simulink library "ConverterLibrary"  (R2026a)
settings: Solver=VariableStepAuto
undefined symbols (not defined in the file or in its folder): DiscIntNeverNeededParam, dspblkCoreblockFVToolHelper, gcbh, gridInverter
libraries: fl_lib x240, nesl_utility x221, ee_lib x208, slpidlib x28, eeGeneralControl x12, simulink x9, eeTransforms x4, simulink_extras x1, eePowerMeasurement x1
(part 2 of 30)

== system ConverterLibrary/Controller/PWM Generators ==
  CLLC PWM Generator : Subsystem  mask(CLLC Resonant Converter PWM Generator){solverMode=Variable-step (continuous), Ts=1e-8, Fbase=100e3, fpuMin=0.6, fpuMax=1.55, pulseWidth=0.5, Tdead=250e-9, Ith=0.5, fpuSrLower=0.97, fpuSrUpper=1.03, Tsr=100e-9, gateVoltageOn=15, gateVoltageOff=0, srGateVoltageOn=15, srGateVoltageOff=0}
      mask prompts: solverMode "Solver mode"; Ts "Sample time (s)"; Fbase "Base (resonant) frequency (Hz)"; fpuMin "Minimum normalized frequency (pu)"; fpuMax "Maximum normalized frequency (pu)"; pulseWidth "Pulse width (fraction of switching period)"; Tdead "Dead time (s)"; Ith "Rectifier current threshold (A)"; fpuSrLower "Resonance band lower edge (pu)"; fpuSrUpper "Resonance band upper edge (pu)"; Tsr "Rectifier turn-on delay (s)"; gateVoltageOn "Gate ON voltage (V)"; gateVoltageOff "Gate OFF voltage (V)"; srGateVoltageOn "Rectifier gate ON voltage (V)"; srGateVoltageOff "Rectifier gate OFF voltage (V)"
      mask help:
      | This block generates full-bridge PWM gate signals with a dead time from a commanded switching frequency, and synchronous rectifier gate signals from the rectifier current.
      |
      | Set the rectifier band lower edge below its upper edge. For a variable-step solver, set Solver mode to Variable-step (continuous). For a fixed-step solver, set Solver mode to Fixed-step (discrete) and set Sample time to a positive value.
      mask init:
      | % Solver mode. Switch every sawtooth ramp in this block between its continuous
      | % and its discrete implementation, and show the sample time only when it is used.
      | pwmGeneratorBlock = gcb;
      | if strcmp(get_param(pwmGeneratorBlock, 'solverMode'), 'Fixed-step (discrete)')
      |     pwmGeneratorRampChoice = 'FixedStep';
      |     pwmGeneratorSampleTimeVisibility = 'on';
      | else
      |     pwmGeneratorRampChoice = 'VariableStep';
      |     pwmGeneratorSampleTimeVisibility = 'off';
      | end
      | 
      | % A block may hold more than one ramp, at any depth, so the ramps are found by the
      | % "Ramp Mode" suffix on their names rather than by one fixed path. The match filter
      | % keeps every variant choice in the search, which is also what silences the
      | % find_system default-variants warning.
      | pwmGeneratorRamps = find_system(pwmGeneratorBlock, ...
      |     'MatchFilter', @Simulink.match.allVariants, 'LookUnderMasks', 'all', ...
      |     'FollowLinks', 'on', 'Regexp', 'on', 'BlockType', 'SubSystem', ...
      |     'Name', 'Ramp Mode$');
      | for pwmGeneratorRampIndex = 1:numel(pwmGeneratorRamps)
      |     set_param(pwmGeneratorRamps{pwmGeneratorRampIndex}, ...
      |         'LabelModeActiveChoice', pwmGeneratorRampChoice);
      | end
      | 
      | % Only the discrete ramp declares a rate, so the sample time is hidden in the
      | % continuous mode. The guard keeps the code silent on a mask still being built.
      | pwmGeneratorMask = Simulink.Mask.get(pwmGeneratorBlock);
      | pwmGeneratorSampleTime = pwmGeneratorMask.getParameter('Ts');
      | if ~isempty(pwmGeneratorSampleTime)
      |     pwmGeneratorSampleTime.Visible = pwmGeneratorSampleTimeVisibility;
      | end
      mask Help: web('CLLCPWMGenerator.html')
      mask TypeOptions solverMode: Variable-step (continuous) | Fixed-step (discrete)
      mask Callback solverMode:
      | % Solver mode. Switch every sawtooth ramp in this block between its continuous
      | % and its discrete implementation, and show the sample time only when it is used.
      | pwmGeneratorBlock = gcb;
      | if strcmp(get_param(pwmGeneratorBlock, 'solverMode'), 'Fixed-step (discrete)')
      |     pwmGeneratorRampChoice = 'FixedStep';
      |     pwmGeneratorSampleTimeVisibility = 'on';
      | else
      |     pwmGeneratorRampChoice = 'VariableStep';
      |     pwmGeneratorSampleTimeVisibility = 'off';
      | end
      | 
      | % A block may hold more than one ramp, at any depth, so the ramps are found by the
      | % "Ramp Mode" suffix on their names rather than by one fixed path. The match filter
      | % keeps every variant choice in the search, which is also what silences the
      | % find_system default-variants warning.
      | pwmGeneratorRamps = find_system(pwmGeneratorBlock, ...
      |     'MatchFilter', @Simulink.match.allVariants, 'LookUnderMasks', 'all', ...
      |     'FollowLinks', 'on', 'Regexp', 'on', 'BlockType', 'SubSystem', ...
      |     'Name', 'Ramp Mode$');
      | for pwmGeneratorRampIndex = 1:numel(pwmGeneratorRamps)
      |     set_param(pwmGeneratorRamps{pwmGeneratorRampIndex}, ...
      |         'LabelModeActiveChoice', pwmGeneratorRampChoice);
      | end
      | 
      | % Only the discrete ramp declares a rate, so the sample time is hidden in the
      | % continuous mode. The guard keeps the code silent on a mask still being built.
      | pwmGeneratorMask = Simulink.Mask.get(pwmGeneratorBlock);
      | pwmGeneratorSampleTime = pwmGeneratorMask.getParameter('Ts');
      | if ~isempty(pwmGeneratorSampleTime)
      |     pwmGeneratorSampleTime.Visible = pwmGeneratorSampleTimeVisibility;
      | end
      mask DialogControl DescTextVar Prompt:
      | This block generates full-bridge PWM gate signals with a dead time from a commanded switching frequency, and synchronous rectifier gate signals from the rectifier current.
      | 
      | Set the rectifier band lower edge below its upper edge. For a variable-step solver, set Solver mode to Variable-step (continuous). For a fixed-step solver, set Solver mode to Fixed-step (discrete) and set Sample time to a positive value.
      mask DialogControl SolverPanel Prompt: Solver Settings
      mask DialogControl SwitchingPanel Prompt: Switching Parameters
      mask DialogControl SyncRectifierPanel Prompt: Synchronous Rectifier
      mask DialogControl GateDrivePanel Prompt: Gate Drive
  Complementary PWM Generator : Subsystem  mask(Complementary PWM Generator){solverMode=Variable-step (continuous), Ts=1e-8, Tdead=100e-9, inputLogicThreshold=0.5, gateVoltageOn=15, gateVoltageOff=0}
      mask prompts: solverMode "Solver mode"; Ts "Sample time (s)"; Tdead "Dead time (s)"; inputLogicThreshold "Input logic threshold (V)"; gateVoltageOn "Gate ON voltage (V)"; gateVoltageOff "Gate OFF voltage (V)"
      mask help:
      | This block splits one PWM signal into a complementary gate pair with a dead time.
      |
      | For a variable-step solver, set Solver mode to Variable-step (continuous). For a fixed-step solver, set Solver mode to Fixed-step (discrete) and set Sample time to a positive value.
      mask init: same as ConverterLibrary/Controller/PWM Generators/CLLC PWM Generator
      mask Help: web('ComplementaryPWMGenerator.html')
      mask TypeOptions solverMode: Variable-step (continuous) | Fixed-step (discrete)
      mask Callback solverMode:
      | % Solver mode. Switch every sawtooth ramp in this block between its continuous
      | % and its discrete implementation, and show the sample time only when it is used.
      | pwmGeneratorBlock = gcb;
      | if strcmp(get_param(pwmGeneratorBlock, 'solverMode'), 'Fixed-step (discrete)')
      |     pwmGeneratorRampChoice = 'FixedStep';
      |     pwmGeneratorSampleTimeVisibility = 'on';
      | else
      |     pwmGeneratorRampChoice = 'VariableStep';
      |     pwmGeneratorSampleTimeVisibility = 'off';
      | end
      | 
      | % A block may hold more than one ramp, at any depth, so the ramps are found by the
      | % "Ramp Mode" suffix on their names rather than by one fixed path. The match filter
      | % keeps every variant choice in the search, which is also what silences the
      | % find_system default-variants warning.
      | pwmGeneratorRamps = find_system(pwmGeneratorBlock, ...
      |     'MatchFilter', @Simulink.match.allVariants, 'LookUnderMasks', 'all', ...
      |     'FollowLinks', 'on', 'Regexp', 'on', 'BlockType', 'SubSystem', ...
      |     'Name', 'Ramp Mode$');
      | for pwmGeneratorRampIndex = 1:numel(pwmGeneratorRamps)
      |     set_param(pwmGeneratorRamps{pwmGeneratorRampIndex}, ...
      |         'LabelModeActiveChoice', pwmGeneratorRampChoice);
      | end
      | 
      | % Only the discrete ramp declares a rate, so the sample time is hidden in the
      | % continuous mode. The guard keeps the code silent on a mask still being built.
      | pwmGeneratorMask = Simulink.Mask.get(pwmGeneratorBlock);
      | pwmGeneratorSampleTime = pwmGeneratorMask.getParameter('Ts');
      | if ~isempty(pwmGeneratorSampleTime)
      |     pwmGeneratorSampleTime.Visible = pwmGeneratorSampleTimeVisibility;
      | end
      mask DialogControl DescTextVar Prompt:
      | This block splits one PWM signal into a complementary gate pair with a dead time.
      | 
      | For a variable-step solver, set Solver mode to Variable-step (continuous). For a fixed-step solver, set Solver mode to Fixed-step (discrete) and set Sample time to a positive value.
      mask DialogControl SolverPanel Prompt: Solver Settings
      mask DialogControl SwitchingPanel Prompt: Switching Parameters
      mask DialogControl GateDrivePanel Prompt: Gate Drive
  DAB PWM Generator : Subsystem  mask(Dual Active Bridge PWM Generator){solverMode=Variable-step (continuous), Ts=1e-8, Fsw=100e3, Tdead=100e-9, primaryGateVoltageOn=15, primaryGateVoltageOff=0, secondaryGateVoltageOn=15, secondaryGateVoltageOff=0}
      mask prompts: solverMode "Solver mode"; Ts "Sample time (s)"; Fsw "Switching frequency (Hz)"; Tdead "Dead time (s)"; primaryGateVoltageOn "Primary bridge gate ON voltage (V)"; primaryGateVoltageOff "Primary bridge gate OFF voltage (V)"; secondaryGateVoltageOn "Secondary bridge gate ON voltage (V)"; secondaryGateVoltageOff "Secondary bridge gate OFF voltage (V)"
      mask help:
      | This block generates dual-active-bridge PWM gate signals with a dead time from a commanded phase shift.
      |
      | For a variable-step solver, set Solver mode to Variable-step (continuous). For a fixed-step solver, set Solver mode to Fixed-step (discrete) and set Sample time to a positive value.
      mask init: same as ConverterLibrary/Controller/PWM Generators/CLLC PWM Generator
      mask Help: web('DABPWMGenerator.html')
      mask TypeOptions solverMode: Variable-step (continuous) | Fixed-step (discrete)
      mask Callback solverMode:
      | % Solver mode. Switch every sawtooth ramp in this block between its continuous
      | % and its discrete implementation, and show the sample time only when it is used.
      | pwmGeneratorBlock = gcb;
      | if strcmp(get_param(pwmGeneratorBlock, 'solverMode'), 'Fixed-step (discrete)')
      |     pwmGeneratorRampChoice = 'FixedStep';
      |     pwmGeneratorSampleTimeVisibility = 'on';
      | else
      |     pwmGeneratorRampChoice = 'VariableStep';
      |     pwmGeneratorSampleTimeVisibility = 'off';
      | end
      | 
      | % A block may hold more than one ramp, at any depth, so the ramps are found by the
      | % "Ramp Mode" suffix on their names rather than by one fixed path. The match filter
      | % keeps every variant choice in the search, which is also what silences the
      | % find_system default-variants warning.
      | pwmGeneratorRamps = find_system(pwmGeneratorBlock, ...
      |     'MatchFilter', @Simulink.match.allVariants, 'LookUnderMasks', 'all', ...
      |     'FollowLinks', 'on', 'Regexp', 'on', 'BlockType', 'SubSystem', ...
      |     'Name', 'Ramp Mode$');
      | for pwmGeneratorRampIndex = 1:numel(pwmGeneratorRamps)
      |     set_param(pwmGeneratorRamps{pwmGeneratorRampIndex}, ...
      |         'LabelModeActiveChoice', pwmGeneratorRampChoice);
      | end
      | 
      | % Only the discrete ramp declares a rate, so the sample time is hidden in the
      | % continuous mode. The guard keeps the code silent on a mask still being built.
      | pwmGeneratorMask = Simulink.Mask.get(pwmGeneratorBlock);
      | pwmGeneratorSampleTime = pwmGeneratorMask.getParameter('Ts');
      | if ~isempty(pwmGeneratorSampleTime)
      |     pwmGeneratorSampleTime.Visible = pwmGeneratorSampleTimeVisibility;
      | end
      mask DialogControl DescTextVar Prompt:
      | This block generates dual-active-bridge PWM gate signals with a dead time from a commanded phase shift.
      | 
      | For a variable-step solver, set Solver mode to Variable-step (continuous). For a fixed-step solver, set Solver mode to Fixed-step (discrete) and set Sample time to a positive value.
      mask DialogControl SolverPanel Prompt: Solver Settings
      mask DialogControl SwitchingPanel Prompt: Switching Parameters
      mask DialogControl GateDrivePanel Prompt: Gate Drive
  Full Bridge PWM Generator : Subsystem  mask(Full Bridge PWM Generator){solverMode=Variable-step (continuous), Ts=1e-8, Fsw=100e3, Tdead=100e-9, gateVoltageOn=15, gateVoltageOff=0}
      mask prompts: solverMode "Solver mode"; Ts "Sample time (s)"; Fsw "Switching frequency (Hz)"; Tdead "Dead time (s)"; gateVoltageOn "Gate ON voltage (V)"; gateVoltageOff "Gate OFF voltage (V)"
      mask help:
      | This block generates full-bridge PWM gate signals with a dead time from a commanded duty cycle.
      |
      | For a variable-step solver, set Solver mode to Variable-step (continuous). For a fixed-step solver, set Solver mode to Fixed-step (discrete) and set Sample time to a positive value.
      mask init: same as ConverterLibrary/Controller/PWM Generators/CLLC PWM Generator
      mask Help: web('FullBridgePWMGenerator.html')
      mask TypeOptions solverMode: Variable-step (continuous) | Fixed-step (discrete)
      mask Callback solverMode:
      | % Solver mode. Switch every sawtooth ramp in this block between its continuous
      | % and its discrete implementation, and show the sample time only when it is used.
      | pwmGeneratorBlock = gcb;
      | if strcmp(get_param(pwmGeneratorBlock, 'solverMode'), 'Fixed-step (discrete)')
      |     pwmGeneratorRampChoice = 'FixedStep';
      |     pwmGeneratorSampleTimeVisibility = 'on';
      | else
      |     pwmGeneratorRampChoice = 'VariableStep';
      |     pwmGeneratorSampleTimeVisibility = 'off';
      | end
      | 
      | % A block may hold more than one ramp, at any depth, so the ramps are found by the
      | % "Ramp Mode" suffix on their names rather than by one fixed path. The match filter
      | % keeps every variant choice in the search, which is also what silences the
      | % find_system default-variants warning.
      | pwmGeneratorRamps = find_system(pwmGeneratorBlock, ...
      |     'MatchFilter', @Simulink.match.allVariants, 'LookUnderMasks', 'all', ...
      |     'FollowLinks', 'on', 'Regexp', 'on', 'BlockType', 'SubSystem', ...
      |     'Name', 'Ramp Mode$');
      | for pwmGeneratorRampIndex = 1:numel(pwmGeneratorRamps)
      |     set_param(pwmGeneratorRamps{pwmGeneratorRampIndex}, ...
      |         'LabelModeActiveChoice', pwmGeneratorRampChoice);
      | end
      | 
      | % Only the discrete ramp declares a rate, so the sample time is hidden in the
      | % continuous mode. The guard keeps the code silent on a mask still being built.
      | pwmGeneratorMask = Simulink.Mask.get(pwmGeneratorBlock);
      | pwmGeneratorSampleTime = pwmGeneratorMask.getParameter('Ts');
      | if ~isempty(pwmGeneratorSampleTime)
      |     pwmGeneratorSampleTime.Visible = pwmGeneratorSampleTimeVisibility;
      | end
      mask DialogControl DescTextVar Prompt:
      | This block generates full-bridge PWM gate signals with a dead time from a commanded duty cycle.
      | 
      | For a variable-step solver, set Solver mode to Variable-step (continuous). For a fixed-step solver, set Solver mode to Fixed-step (discrete) and set Sample time to a positive value.
      mask DialogControl SolverPanel Prompt: Solver Settings
      mask DialogControl SwitchingPanel Prompt: Switching Parameters
      mask DialogControl GateDrivePanel Prompt: Gate Drive
  Half Bridge PWM Generator : Subsystem  mask(Half Bridge PWM Generator){solverMode=Variable-step (continuous), Ts=1e-8, Fsw=100e3, Tdead=100e-9, gateVoltageOn=15, gateVoltageOff=0}
      mask prompts: solverMode "Solver mode"; Ts "Sample time (s)"; Fsw "Switching frequency (Hz)"; Tdead "Dead time (s)"; gateVoltageOn "Gate ON voltage (V)"; gateVoltageOff "Gate OFF voltage (V)"
      mask help:
      | This block generates half-bridge PWM gate signals with a dead time from a commanded duty cycle.
      |
      | For a variable-step solver, set Solver mode to Variable-step (continuous). For a fixed-step solver, set Solver mode to Fixed-step (discrete) and set Sample time to a positive value.
      mask init: same as ConverterLibrary/Controller/PWM Generators/CLLC PWM Generator
      mask Help: web('HalfBridgePWMGenerator.html')
      mask TypeOptions solverMode: Variable-step (continuous) | Fixed-step (discrete)
      mask Callback solverMode:
      | % Solver mode. Switch every sawtooth ramp in this block between its continuous
      | % and its discrete implementation, and show the sample time only when it is used.
      | pwmGeneratorBlock = gcb;
      | if strcmp(get_param(pwmGeneratorBlock, 'solverMode'), 'Fixed-step (discrete)')
      |     pwmGeneratorRampChoice = 'FixedStep';
      |     pwmGeneratorSampleTimeVisibility = 'on';
      | else
      |     pwmGeneratorRampChoice = 'VariableStep';
      |     pwmGeneratorSampleTimeVisibility = 'off';
      | end
      | 
      | % A block may hold more than one ramp, at any depth, so the ramps are found by the
      | % "Ramp Mode" suffix on their names rather than by one fixed path. The match filter
      | % keeps every variant choice in the search, which is also what silences the
      | % find_system default-variants warning.
      | pwmGeneratorRamps = find_system(pwmGeneratorBlock, ...
      |     'MatchFilter', @Simulink.match.allVariants, 'LookUnderMasks', 'all', ...
      |     'FollowLinks', 'on', 'Regexp', 'on', 'BlockType', 'SubSystem', ...
      |     'Name', 'Ramp Mode$');
      | for pwmGeneratorRampIndex = 1:numel(pwmGeneratorRamps)
      |     set_param(pwmGeneratorRamps{pwmGeneratorRampIndex}, ...
      |         'LabelModeActiveChoice', pwmGeneratorRampChoice);
      | end
      | 
      | % Only the discrete ramp declares a rate, so the sample time is hidden in the
      | % continuous mode. The guard keeps the code silent on a mask still being built.
      | pwmGeneratorMask = Simulink.Mask.get(pwmGeneratorBlock);
      | pwmGeneratorSampleTime = pwmGeneratorMask.getParameter('Ts');
      | if ~isempty(pwmGeneratorSampleTime)
      |     pwmGeneratorSampleTime.Visible = pwmGeneratorSampleTimeVisibility;
      | end
      mask DialogControl DescTextVar Prompt:
      | This block generates half-bridge PWM gate signals with a dead time from a commanded duty cycle.
      | 
      | For a variable-step solver, set Solver mode to Variable-step (continuous). For a fixed-step solver, set Solver mode to Fixed-step (discrete) and set Sample time to a positive value.
      mask DialogControl SolverPanel Prompt: Solver Settings
      mask DialogControl SwitchingPanel Prompt: Switching Parameters
      mask DialogControl GateDrivePanel Prompt: Gate Drive
  LLC PWM Generator : Subsystem  mask(LLC Resonant Converter PWM Generator){solverMode=Variable-step (continuous), Ts=1e-8, Fbase=100e3, fpuMin=0.5, fpuMax=2, pulseWidth=0.5, Tdead=100e-9, gateVoltageOn=15, gateVoltageOff=0}
      mask prompts: solverMode "Solver mode"; Ts "Sample time (s)"; Fbase "Base (resonant) frequency (Hz)"; fpuMin "Minimum normalized frequency (pu)"; fpuMax "Maximum normalized frequency (pu)"; pulseWidth "Pulse width (fraction of switching period)"; Tdead "Dead time (s)"; gateVoltageOn "Gate ON voltage (V)"; gateVoltageOff "Gate OFF voltage (V)"
      mask help:
      | This block generates full-bridge PWM gate signals with a dead time from a commanded switching frequency.
      |
      | For a variable-step solver, set Solver mode to Variable-step (continuous). For a fixed-step solver, set Solver mode to Fixed-step (discrete) and set Sample time to a positive value.
      mask init: same as ConverterLibrary/Controller/PWM Generators/CLLC PWM Generator
      mask Help: web('LLCPWMGenerator.html')
      mask TypeOptions solverMode: Variable-step (continuous) | Fixed-step (discrete)
      mask Callback solverMode:
      | % Solver mode. Switch every sawtooth ramp in this block between its continuous
      | % and its discrete implementation, and show the sample time only when it is used.
      | pwmGeneratorBlock = gcb;
      | if strcmp(get_param(pwmGeneratorBlock, 'solverMode'), 'Fixed-step (discrete)')
      |     pwmGeneratorRampChoice = 'FixedStep';
      |     pwmGeneratorSampleTimeVisibility = 'on';
      | else
      |     pwmGeneratorRampChoice = 'VariableStep';
      |     pwmGeneratorSampleTimeVisibility = 'off';
      | end
      | 
      | % A block may hold more than one ramp, at any depth, so the ramps are found by the
      | % "Ramp Mode" suffix on their names rather than by one fixed path. The match filter
      | % keeps every variant choice in the search, which is also what silences the
      | % find_system default-variants warning.
      | pwmGeneratorRamps = find_system(pwmGeneratorBlock, ...
      |     'MatchFilter', @Simulink.match.allVariants, 'LookUnderMasks', 'all', ...
      |     'FollowLinks', 'on', 'Regexp', 'on', 'BlockType', 'SubSystem', ...
      |     'Name', 'Ramp Mode$');
      | for pwmGeneratorRampIndex = 1:numel(pwmGeneratorRamps)
      |     set_param(pwmGeneratorRamps{pwmGeneratorRampIndex}, ...
      |         'LabelModeActiveChoice', pwmGeneratorRampChoice);
      | end
      | 
      | % Only the discrete ramp declares a rate, so the sample time is hidden in the
      | % continuous mode. The guard keeps the code silent on a mask still being built.
      | pwmGeneratorMask = Simulink.Mask.get(pwmGeneratorBlock);
      | pwmGeneratorSampleTime = pwmGeneratorMask.getParameter('Ts');
      | if ~isempty(pwmGeneratorSampleTime)
      |     pwmGeneratorSampleTime.Visible = pwmGeneratorSampleTimeVisibility;
      | end
      mask DialogControl DescTextVar Prompt:
      | This block generates full-bridge PWM gate signals with a dead time from a commanded switching frequency.
      | 
      | For a variable-step solver, set Solver mode to Variable-step (continuous). For a fixed-step solver, set Solver mode to Fixed-step (discrete) and set Sample time to a positive value.
      mask DialogControl SolverPanel Prompt: Solver Settings
      mask DialogControl SwitchingPanel Prompt: Switching Parameters
      mask DialogControl GateDrivePanel Prompt: Gate Drive

== system ConverterLibrary/Controller/Power Factor Correction Converters ==
  Boost PFC Controller : Subsystem  mask(Boost PFC Controller){outputSelect=PWM Signal, cntrlSelect=PI controller (Continuous), VacRMS=230, VbaseDC=400, Pbase=1000, PrefPu=1, iRefPeakMaxPu=1.3, Fsw=65000, Ts=7.6923e-8, gateVoltageOn=15, gateVoltageOff=0, KpVoltage=1.0392, KiVoltage=11.3097, TsVoltage=7.6923e-6, KpCurrent=0.2602, KiCurrent=3068.1596, dutyMax=0.9935, dutyMin=0.0065, TsCurrent=1.5385e-6}
      mask prompts: outputSelect "Output"; cntrlSelect "Controller type"; VacRMS "Nominal line voltage, RMS (V)"; VbaseDC "Regulated bus voltage (V)"; Pbase "Rated power (W)"; PrefPu "Power command (pu)"; iRefPeakMaxPu "Peak current limit (pu)"; Fsw "Switching frequency (Hz)"; Ts "Modulator sample time (s)"; gateVoltageOn "Gate voltage, on (V)"; gateVoltageOff "Gate voltage, off (V)"; KpVoltage "Voltage-loop proportional gain (pu)"; KiVoltage "Voltage-loop integral gain (pu/s)"; TsVoltage "Voltage-loop sample time (s)"; KpCurrent "Current-loop proportional gain (pu)"; KiCurrent "Current-loop integral gain (pu/s)"; dutyMax "Maximum duty cycle"; dutyMin "Minimum duty cycle"; TsCurrent "Current-loop sample time (s)"
      mask help: Average-current-mode power factor correction controller for the single-leg boost PFC. Regulates the DC bus voltage while shaping the AC line current sinusoidal and in phase, for near-unity power factor. Offers PI controllers in continuous or discrete form, with selectable duty cycle or PWM gate signal output.
      mask init:
      | VbaseAC = sqrt(2)*VacRMS;
      | IbaseAC = 2*Pbase/VbaseAC;
      | VacPeakPuDC = VbaseAC/VbaseDC;
      | 
      | boostPFCControllerMaskInit(gcb);
      mask Help: web('BoostPFCController.html')
      mask TypeOptions outputSelect: Duty Cycle | PWM Signal
      mask Callback outputSelect: boostPFCControllerMaskInit(gcb);
      mask TypeOptions cntrlSelect: PI controller (Continuous) | PI controller (Discrete)
      mask Callback cntrlSelect: boostPFCControllerMaskInit(gcb);
      mask DialogControl ConverterPanel Prompt: Boost PFC Controller Parameters
      mask DialogControl VoltageLoopPanel Prompt: Voltage Controller
      mask DialogControl CurrentLoopPanel Prompt: Current Controller
  Interleaved Boost PFC Controller : Subsystem  mask(Interleaved Boost PFC Controller){outputSelect=PWM Signal, cntrlSelect=PI controller (Continuous), VacRMS=230, VbaseDC=400, Pbase=2000, numberOfLegs=2, PrefPu=1, iRefPeakMaxPu=1.3, Fsw=65000, Ts=7.6923e-8, gateVoltageOn=15, gateVoltageOff=0, KpVoltage=1.0392, KiVoltage=11.3097, TsVoltage=7.6923e-6, KpCurrent=0.2602, KiCurrent=3068.1596, dutyMax=0.9935, dutyMin=0.0065, TsCurrent=1.5385e-6, KpBalance=0.1041, KiBalance=245.4528, dutyBalanceMax=0.1}
      mask prompts: outputSelect "Output"; cntrlSelect "Controller type"; VacRMS "Nominal line voltage, RMS (V)"; VbaseDC "Regulated bus voltage (V)"; Pbase "Rated power (W)"; numberOfLegs "Number of interleaved legs"; PrefPu "Power command (pu)"; iRefPeakMaxPu "Peak current-reference limit (pu)"; Fsw "Switching frequency (Hz)"; Ts "Modulator sample time (s)"; gateVoltageOn "Gate voltage, on (V)"; gateVoltageOff "Gate voltage, off (V)"; KpVoltage "Voltage-loop proportional gain (pu)"; KiVoltage "Voltage-loop integral gain (pu/s)"; TsVoltage "Voltage-loop sample time (s)"; KpCurrent "Current-loop proportional gain (pu)"; KiCurrent "Current-loop integral gain (pu/s)"; dutyMax "Maximum duty cycle"; dutyMin "Minimum duty cycle"; TsCurrent "Current-loop sample time (s)"; KpBalance "Balance-loop proportional gain (pu)"; KiBalance "Balance-loop integral gain (pu/s)"; dutyBalanceMax "Balance-loop duty trim limit"
      mask help: Average-current-mode power factor correction controller for the interleaved boost PFC. Regulates the DC bus voltage while shaping the AC line current sinusoidal and in phase, for near-unity power factor. One shared control serves all legs, with phase-shifted carriers and a differential loop that balances the leg currents. Offers PI controllers in continuous or discrete form, with selectable duty cycle or PWM gate signal output.
      mask init:
      | VbaseAC = sqrt(2)*VacRMS;
      | IbaseAC = 2*Pbase/VbaseAC;
      | VacPeakPuDC = VbaseAC/VbaseDC;
      | 
      | interleavedPFCControllerMaskInit(gcb);
      mask Help: web('InterleavedBoostPFCController.html')
      mask TypeOptions outputSelect: Duty Cycle | PWM Signal
      mask Callback outputSelect: interleavedPFCControllerMaskInit(gcb);
      mask TypeOptions cntrlSelect: PI controller (Continuous) | PI controller (Discrete)
      mask Callback cntrlSelect: interleavedPFCControllerMaskInit(gcb);
      mask DialogControl ConverterPanel Prompt: Interleaved Boost PFC Controller Parameters
      mask DialogControl VoltageLoopPanel Prompt: Voltage Controller
      mask DialogControl CurrentLoopPanel Prompt: Current Controller
      mask DialogControl CurrentBalancePanel Prompt: Current Balance Controller
  Totem-Pole Boost PFC Controller : Subsystem  mask(Totem-Pole Boost PFC Current-Mode Controller){outputSelect=PWM Signal, cntrlSelect=PI controller (Continuous), VacRMS=230, VbaseDC=400, Pbase=3000, Fsw=100000, Fline=50, fastLegDeadTime=1e-07, slowLegTurnOnDelay=0.0001, PrefPu=0.5, iRefPeakMaxPu=1.2, gateVoltageOn=15, gateVoltageOff=0, KpVoltage=1.0392, KiVoltage=11.3097, TsVoltage=5e-06, KpCurrent=0.2602, KiCurrent=4720.2456, dutyMax=1, dutyMin=0, TsCurrent=1e-06}
      mask prompts: outputSelect "Output mode"; cntrlSelect "Controller type"; VacRMS "Nominal AC voltage (V RMS)"; VbaseDC "Nominal DC voltage (V)"; Pbase "Nominal power (W)"; Fsw "Switching frequency (Hz)"; Fline "Line frequency (Hz)"; fastLegDeadTime "Fast-leg dead time (s)"; slowLegTurnOnDelay "Slow-leg turn-on delay (s)"; PrefPu "Feedforward power (pu)"; iRefPeakMaxPu "Peak current limit (pu)"; gateVoltageOn "Gate ON voltage (V)"; gateVoltageOff "Gate OFF voltage (V)"; KpVoltage "Proportional gain (pu)"; KiVoltage "Integral gain (pu/s)"; TsVoltage "Sample time (s)"; KpCurrent "Proportional gain (pu)"; KiCurrent "Integral gain (pu/s)"; dutyMax "Maximum duty cycle"; dutyMin "Minimum duty cycle"; TsCurrent "Sample time (s)"
      mask help: Average-current-mode power factor correction controller for the totem-pole boost PFC. Regulates the DC bus voltage while shaping the AC line current sinusoidal and in phase, for near-unity power factor. Offers PI controllers in continuous or discrete form, with selectable duty cycle or PWM gate signal output.
      mask init:
      | VbaseAC = sqrt(2)*VacRMS;
      | IbaseAC = 2*Pbase/VbaseAC;
      | VacPeakPuDC = VbaseAC/VbaseDC;
      | 
      | totemPolePFCControllerMaskInit(gcb);
      mask Help: web('TotemPoleBoostPFCController.html')
      mask TypeOptions outputSelect: Duty Cycle | PWM Signal
      mask Callback outputSelect: totemPolePFCControllerMaskInit(gcb);
      mask TypeOptions cntrlSelect: PI controller (Continuous) | PI controller (Discrete)
      mask Callback cntrlSelect: totemPolePFCControllerMaskInit(gcb);
      mask DialogControl ConverterPanel Prompt: Totem-Pole Boost PFC Controller Parameters
      mask DialogControl VoltageLoopPanel Prompt: Voltage Controller
      mask DialogControl CurrentLoopPanel Prompt: Current Controller

== system ConverterLibrary/Controller/Soft-Switching Converters ==
  CLLC Controller : Subsystem  mask(CLLC Resonant Converter Voltage Controller){controllerDomain=Continuous, resFreq=100000, ratedPower=10000, Fmin=0.6, Fmax=2.015, Tdead=2.5e-07, VdcValue=400, Kpv=11, Kiv=5500, Kid=0, IdcMax=2.5, IdcMin=-2.5, cntrlSelect=PI controller, Kc=1, numSdomain=[1 1463 1794700], denSdomain=[1 2748.6 0], numZdomain=[1 -1.9985 0.9985], denZdomain=[1 -1.9973 0.9973], Kp=3.5, Ki=5, Ith=0.5, Ibw=300000, vcoSelect=Constant rate, vcoGain=1, vcoGainVec=[1 1.2], pwmSampleTime=1.25e-07, TsVoltage=1e-06, TsCurrent=1e-06}
      mask prompts: controllerDomain "Controller time domain"; resFreq "Resonant frequency"; ratedPower "Rated power (W)"; Fmin "Minimum operating frequency (pu)"; Fmax "Maximum operating frequency (pu)"; Tdead "dead time (s)"; VdcValue "Nominal DC bus voltage"; Kpv "Proportional gain"; Kiv "Integrator gain"; Kid "Differentiator gain"; IdcMax "Maximum output current (pu)"; IdcMin "Minimum output current (put)"; cntrlSelect "Controller type"; Kc "Compensator gain"; numSdomain "Numerator (S domain)"; denSdomain "Denominator (S domain)"; numZdomain "Numerator (Z domain)"; denZdomain "Denominator (Z domain)"; Kp "Proportional gain"; Ki "Integrator gain (Ki)"; Ith "Current threshold (A)"; Ibw "Measurement bandwidth (Hz)"; vcoSelect "Voltage-controlled oscillator type"; vcoGain "VCO gain rate (V/perunit frequency)"; vcoGainVec "VCO gain [g1 g2]  (V/perunit frequency)"; pwmSampleTime "PWM sample time (s)"; TsVoltage "Sample time (s)"; TsCurrent "Sample time (s)"
      mask help: The CLLC resonant converter controller offers four controller options: you can choose between a two-pole, two-zero (2P2Z) compensator and a PI controller, each available in continuous or discrete form. The controller also provides three options for selecting the voltage-controlled oscillator (VCO) gain.
      mask init:
      | % Rate of the block that gates the voltage loop. A discrete voltage controller cannot
      | % inherit a continuous rate, so that block is given the controller rate.
      | gatingSampleTime = gatingSampleTimeForControllerType(controllerDomain, TsVoltage);
      | 
      | cllcControllerMaskInitialization(gcb);
      mask Help: web('CLLCController.html')
      mask TypeOptions controllerDomain: Continuous | Discrete
      mask Callback controllerDomain: selectCLLCControllerVariants(gcb);
      mask TypeOptions cntrlSelect: 2P2Z compensator | PI controller
      mask Callback cntrlSelect: selectCLLCMaskController(gcb);
      mask TypeOptions vcoSelect: Constant rate | Two rate
      mask Callback vcoSelect: selectCLLCControllerMaskVCO(gcb);
      mask DialogControl ParameterGroupVar Prompt: LLC Controller Parameters
      mask DialogControl Container6 Prompt: Voltage Controller Parameters
      mask DialogControl Container3 Prompt: Current Controller Parameters
      mask DialogControl Container5 Prompt: Synchronous rectitifer
      mask DialogControl Container4 Prompt: Voltage-Controlled Oscillator Parameters
      mask DialogControl Container7 Prompt: PWM Generator
  DAB Controller (SPS) : Subsystem  mask(Dual Active Bridge Phase-Shift Controller){outputSelect=Gate Signals, cntrlSelect=PI controller (Continuous), Vbase=525, Pbase=10000, Fsw=100000, Tdead=4.3943e-7, primaryGateVoltage=15, secondaryGateVoltage=15, Ts=1e-07, phaseShiftMax=pi/2, phaseShiftMin=-pi/2, Kp=0.0008, Ki=600, Kpv=0.0075, Kiv=600}
      mask prompts: outputSelect "Output mode"; cntrlSelect "Controller type"; Vbase "Nominal output voltage (V)"; Pbase "Nominal power (W)"; Fsw "Switching frequency (Hz)"; Tdead "Dead time (s)"; primaryGateVoltage "Primary gate voltage (V)"; secondaryGateVoltage "Secondary gate voltage (V)"; Ts "Sample time (s)"; phaseShiftMax "Max phase shift (rad)"; phaseShiftMin "Min phase shift (rad)"; Kp "Proportional gain (current loop)"; Ki "Integral gain (current loop)"; Kpv "Proportional gain (voltage loop)"; Kiv "Integral gain (voltage loop)"
      mask help:
      | Phase-shift controller for the dual-active-bridge converter, in constant-current or constant-voltage mode. The CCCV input selects which loop runs: CC regulates Imeas against a current reference on Ref, normalized on the base current Pbase/Vbase; CV regulates Vmeas against a voltage reference on Ref, normalized on Vbase. Either PI drives the bridge-to-bridge phase shift, limited by phaseShiftMin and phaseShiftMax. Offers PI controllers in continuous or discrete form, with selectable phase shift or gate signal output.
      |
      | Outputs G1 and G2 are the primary and secondary bridge gate vectors, at the levels set by primaryGateVoltage and secondaryGateVoltage. In Phase Shift (rad) mode both outputs instead carry the phase shift itself, for use with an averaged plant.
      mask init:
      | dabControllerMaskInit(gcb);
      mask Help: web('DABController.html')
      mask TypeOptions outputSelect: Gate Signals | Phase Shift (rad)
      mask Callback outputSelect: selectDABControllerOutputMode(gcb);
      mask TypeOptions cntrlSelect: PI controller (Continuous) | PI controller (Discrete)
      mask Callback cntrlSelect: selectDABControllerType(gcb);
      mask DialogControl Container5 Prompt: DAB Converter Parameter
      mask DialogControl ControllerPanel Prompt: Current Controller
      mask DialogControl VoltageLoopPanel Prompt: Voltage Controller
  LLC Voltage Controller : Subsystem  mask(LLC Resonant Converter Voltage Controller){resFreq=100000, Fmin=0.8, Fmax=2, Tdead=2.5e-07, cntrlSelect=Compensator (Continuous S domain), VdcValue=400, Kc=1, numSdomain=[1 5653.2 5.6475e+07], denSdomain=[1 84698 0], numZdomain=[1 -1.9946 0.9946], denZdomain=[1 -1.9188 0.9188], Kp=3.5, Ki=5, TsController=1e-06, vcoSelect=Constant rate, vcoGain=1, vcoGainVec=[1 1], pwmSampleTime=1e-7}
      mask prompts: resFreq "Resonant frequency"; Fmin "Minimum operating frequency (pu)"; Fmax "Maximum operating frequency (pu)"; Tdead "dead time (s)"; cntrlSelect "Controller type"; VdcValue "Nominal DC bus voltage"; Kc "Compensator gain"; numSdomain "Numerator (S domain)"; denSdomain "Denominator (S domain)"; numZdomain "Numerator (Z domain)"; denZdomain "Denominator (Z domain)"; Kp "Proportional gain"; Ki "Integrator gain (Ki)"; TsController "Sample time"; vcoSelect "Voltage-controlled oscillator type"; vcoGain "VCO gain rate (V/perunit frequency)"; vcoGainVec "VCO gain [g1 g2]  (V/perunit frequency)"; pwmSampleTime "PWM sample time (s)"
      mask help: The LLC resonant converter controller offers four controller options: you can choose between a two-pole, two-zero (2P2Z) compensator and a PI controller, each available in continuous or discrete form. The controller also provides three options for selecting the voltage-controlled oscillator (VCO) gain.
      mask init:
      | llcControllerMaskInitialization(gcb);
      | 
      | % The PWM carrier follows the controller type and is not asked for on this dialog.
      | applyDerivedPWMCarrier(gcb, 'LLC PWM Generator', 'pwmSampleTime');
      settings: PortSchema="{\"entries\":[{\"content\":{\"sides\":[{\"content\":{\"connectorIds\":[\"In1\"]},\"type\":\"ConnectorPlacement.EquallySpacedRectSide\",\"uuid\":\"84c754b2-b57a-4f64-aca2-bece432afc0f\"},{\"content\":{\"connectorIds\":[\"Out1\"],\"side\":\"RIGHT\"},\"type\":\"ConnectorPlacement.EquallySpacedRectSide\",\"uuid\":\"31c81acd-cffa-43b1-9c63-1fa24393f775\"},{\"content\":{\"connectorIds\":[\"In2\"],\"side\":\"TOP\"},\"type\":\"ConnectorPlacement.EquallySpacedRectSide\",\"uuid\":\"46f30af2-e083-46a8-989c-736cac31dc66\"}]},\"type\":\"ConnectorPlacement.EquallySpacedConnector\",\"uuid\":\"410fd2ee-b5f6-4e6f-ac81-4da5eb330e7f\"}],\"packageUris\":[\"http://schema.mathworks.com/mf0/Connector/R2020b\"],\"version\":\"1.0\"}"
      mask Help: web('LLCController.html')
      mask TypeOptions cntrlSelect: Compensator (Continuous S domain) | Compensator (Discrete Z domain) | PI controller (Continuous) | PI controller (Discrete)
      mask Callback cntrlSelect:
      | selectLLCMaskController(gcb);
      | applyDerivedPWMCarrier(gcb, 'LLC PWM Generator', 'pwmSampleTime');
      mask TypeOptions vcoSelect: Constant rate | Two rate
      mask Callback vcoSelect: selectLLCControllerMaskVCO(gcb);
      mask DialogControl ParameterGroupVar Prompt: LLC Controller Parameters
      mask DialogControl Container3 Prompt: Controller Parameters
      mask DialogControl Container4 Prompt: Voltage-Controlled Oscillator Parameters
      mask DialogControl Container5 Prompt: PWM Generator

== system ConverterLibrary/Power Converter Plant/Non-Isolated DC-DC Converters ==
  Non-Isolated DC-DC Converter : Subsystem  mask(Non-Isolated DC-DC Converter){modelOption=Synchronous Boost, ratedPower=1500, ratedPower_unit=W, Vin=200, Vin_unit=V, Vout=400, Vout_unit=V, Fsw=100000, Fsw_unit=Hz, L=4.356e-4, L_unit=H, RL=0.05, RL_unit=Ohm, C=1.8651e-4, C_unit=F, Rco=0.02, Rco_unit=Ohm, Vco=320, Vco_unit=V, switchDeviceOption=Ideal Switch, RdsOn=0.02, RdsOn_unit=Ohm, GdsOff=1e-05, GdsOff_unit=1/Ohm, Vth=0.5, Vth_unit=V, VfBody=2.04, VfBody_unit=V, RdBody=0.004, RdBody_unit=Ohm, GdBody=1e-6, GdBody_unit=1/Ohm, diodeDeviceOption=Ideal Diode, Vf=0.5, Vf_unit=V, Rd=0.01, Rd_unit=Ohm, Gd=1e-05, Gd_unit=1/Ohm, simTemp=25, simTemp_unit=degC}
      mask prompts: modelOption "Topology"; ratedPower "Rated power"; Vin "Input voltage"; Vout "Output voltage"; Fsw "Switching frequency"; L "Inductance"; RL "Inductor resistance"; C "Output capacitance"; Rco "Capacitor ESR"; Vco "Initial output capacitor voltage"; switchDeviceOption "Main switch device"; RdsOn "On-state resistance"; GdsOff "Off-state conductance"; Vth "Threshold voltage"; VfBody "Body diode forward voltage"; RdBody "Body diode on resistance"; GdBody "Body diode off conductance"; diodeDeviceOption "Diode device"; Vf "Diode forward voltage"; Rd "Diode on resistance"; Gd "Diode off conductance"; simTemp "Simulation temperature"
      mask help: Buck, Boost, or Buck-Boost DC-DC converter with optional synchronous rectification
      mask init:
      | %% Unit conversion: convert displayed values to base SI units
      | convMap = containers.Map( ...
      |     {'W','kW','MW','V','kV','mV','F','mF','uF','nF','pF', ...
      |      'H','mH','uH','nH','Ohm','kOhm','mOhm','S','mS','1/Ohm', ...
      |      'Hz','kHz','MHz'}, ...
      |     {1, 1e3, 1e6, 1, 1e3, 1e-3, 1, 1e-3, 1e-6, 1e-9, 1e-12, ...
      |      1, 1e-3, 1e-6, 1e-9, 1, 1e3, 1e-3, 1, 1e-3, 1, ...
      |      1, 1e3, 1e6});
      | 
      | ratedPower_SI = ratedPower * convMap(ratedPower_unit);
      | Vin_SI = Vin * convMap(Vin_unit);
      | Vout_SI = Vout * convMap(Vout_unit);
      | Fsw_SI = Fsw * convMap(Fsw_unit);
      | L_SI = L * convMap(L_unit);
      | RL_SI = RL * convMap(RL_unit);
      | C_SI = C * convMap(C_unit);
      | Rco_SI = Rco * convMap(Rco_unit);
      | Vco_SI = Vco * convMap(Vco_unit);
      | RdsOn_SI = RdsOn * convMap(RdsOn_unit);
      | GdsOff_SI = GdsOff * convMap(GdsOff_unit);
      | Vth_SI = Vth * convMap(Vth_unit);
      | Vf_SI = Vf * convMap(Vf_unit);
      | Rd_SI = Rd * convMap(Rd_unit);
      | Gd_SI = Gd * convMap(Gd_unit);
      | VfBody_SI = VfBody * convMap(VfBody_unit);
      | RdBody_SI = RdBody * convMap(RdBody_unit);
      | GdBody_SI = GdBody * convMap(GdBody_unit);
      | 
      | %% Simulation temperature
      | % Temperature is an offset unit (K = degC + 273.15), so it cannot use convMap.
      | % simTemp_K is read by the thermal MOSFET junction target and Temperature Source,
      | % and by the tabulated diode device temperature.
      | if strcmp(simTemp_unit, 'degC')
      |     simTemp_K = simTemp + 273.15;
      | else
      |     simTemp_K = simTemp;
      | end
      | 
      | %% Apply variant selection
      | selectDCDCModelOption(gcb);
      settings: CopyFcn="set_param(gcbh,\"LinkStatus\",\"none\");"  PortSchema="{\"entries\":[{\"content\":{\"sides\":[{\"content\":{\"connectorIds\":[\"LConn1\",\"LConn2\"]},\"type\":\"ConnectorPlacement.EquallySpacedRectSide\",\"uuid\":\"902a8dfc-7104-4c05-856d-94df839e3447\"},{\"content\":{\"connectorIds\":[\"RConn1\",\"RConn2\"],\"side\":\"RIGHT\"},\"type\":\"ConnectorPlacement.EquallySpacedRectSide\",\"uuid\":\"60097652-723c-4c8b-adb2-e2e896cce9b8\"},{\"content\":{\"connectorIds\":[\"In1\",\"Out1\"],\"side\":\"TOP\"},\"type\":\"ConnectorPlacement.EquallySpacedRectSide\",\"uuid\":\"37713e19-e822-434b-b66d-56986e674464\"}]},\"type\":\"ConnectorPlacement.EquallySpacedConnector\",\"uuid\":\"e0b4e08f-2e15-4704-9b91-0fcfb097a2d4\"}],\"packageUris\":[\"http://schema.mathworks.com/mf0/Connector/R2020b\"],\"version\":\"1.0\"}"
      mask Help: web('NonIsolatedDCDC.html')
      mask TypeOptions modelOption: Buck | Synchronous Buck | Boost | Synchronous Boost | Buck-Boost | Synchronous Buck-Boost
      mask Callback modelOption: selectDCDCModelOption(gcb);
      mask TypeOptions ratedPower_unit: W | kW | MW
      mask TypeOptions Vin_unit: V | mV | kV
      mask TypeOptions Vout_unit: V | mV | kV
      mask TypeOptions Fsw_unit: Hz | kHz | MHz
      mask TypeOptions L_unit: H | mH | uH | nH
      mask TypeOptions RL_unit: Ohm | mOhm
      mask TypeOptions C_unit: F | mF | uF | nF | pF
      mask TypeOptions Rco_unit: Ohm | mOhm
      mask TypeOptions Vco_unit: V | kV | mV
      mask TypeOptions switchDeviceOption: Ideal Switch | MOSFET (Ideal, Switching) with Thermal
      mask Callback switchDeviceOption: selectDCDCMainSwitch(gcb);
      mask TypeOptions RdsOn_unit: Ohm | mOhm
      mask TypeOptions GdsOff_unit: 1/Ohm | S
      mask TypeOptions Vth_unit: V | mV
      mask TypeOptions VfBody_unit: V | mV
      mask TypeOptions RdBody_unit: Ohm | mOhm
      mask TypeOptions GdBody_unit: 1/Ohm | S
      mask TypeOptions diodeDeviceOption: Ideal Diode | Tabulated Diode
      mask Callback diodeDeviceOption: selectDCDCDiodeDevice(gcb);
      mask TypeOptions Vf_unit: V | mV
      mask TypeOptions Rd_unit: Ohm | mOhm
      mask TypeOptions Gd_unit: 1/Ohm | S
      mask TypeOptions simTemp_unit: degC | K
      mask DialogControl DC_DCConverterParameters Prompt: DC-DC Converter Parameters
      mask DialogControl SwitchDevice Prompt: Switch Device
      mask DialogControl openMOSFETMask Prompt: Open MOSFET block mask
      mask DialogControl openMOSFETMask Callback: openDCDCMOSFETMask(gcb);
      mask DialogControl DiodeDevice Prompt: Diode Device
      mask DialogControl openDiodeMask Prompt: Open Diode block mask
      mask DialogControl openDiodeMask Callback: openDCDCDiodeMask(gcb);
      mask DialogControl ExportPanel Prompt: Export to Unmasked Subsystem
      mask DialogControl ExportInfo Prompt: To customize the converter, export it as an unmasked subsystem with the active variant flattened - a standalone, fully-editable circuit plus a parameter file. Requires the "Variant Manager for Simulink" add-on.
      mask DialogControl exportToModel Prompt: Export
      mask DialogControl exportToModel Callback: exportConverterModelFromMask(gcb);
      mask Display:
      | topology = get_param(gcb, 'modelOption');
      | if strcmp(topology, 'Buck')
      |     image('BuckDiodeIcon.svg');
      | elseif strcmp(topology, 'Synchronous Buck')
      |     image('BuckSyncMOSIcon.svg');
      | elseif strcmp(topology, 'Boost')
      |     image('BoostDiodeIcon.svg');
      | elseif strcmp(topology, 'Synchronous Boost')
      |     image('BoostSyncMOSIcon.svg');
      | elseif strcmp(topology, 'Buck-Boost')
      |     image('BuckBoostDiodeIcon.svg');
      | else
      |     image('BuckBoostSyncMOSIcon.svg');
      | end
